simulink model "title4"  (R2024b)
settings: Solver=VariableStepAuto  StartTime=0.0  StopTime=2  RelTol=1e-3
libraries: fl_lib x10, spsSeriesRLCBranchLib x6, nesl_utility x5, spsThyristorLib x4, spsVoltageMeasurementLib x4, spsCurrentMeasurementLib x2, spsDiodeLib x2, spsMosfetLib x2, simulink x2, spsGroundLib x1, slpidlib x1, eePwmGenerator x1
settings Model: VariantFading=off  Creator=Abdal  LastModifiedBy=Abdal
settings DebuggingCC: AlgebraicLoopMsg=none

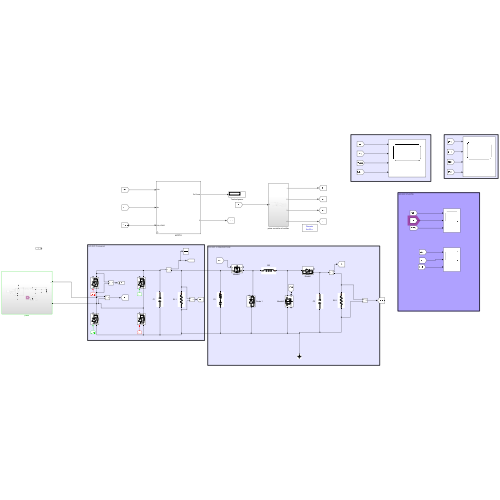
[thumbnail: Simulink's stored preview of the top-level diagram]
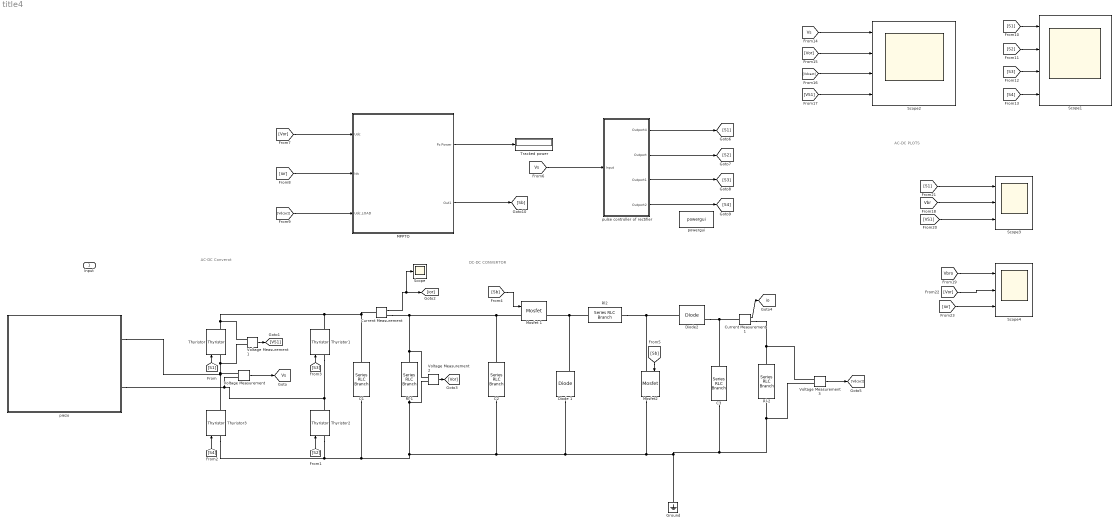
== system title4 ==
  note: AC-DC PLOTS
  note: DC-DC CONVERTOR
  note: AC-DC Converot
  Input : Inport
  C1 : spsSeriesRLCBranchLib/Series RLC Branch  LConnTagsString=__new0  RConnTagsString=__new0  BranchType=C  Resistance=1  Inductance=1e-3  SetiL0=off  InitialCurrent=0  Capacitance=4500e-6  Setx0=off  InitialVoltage=0  Measurements=None
  C2 : spsSeriesRLCBranchLib/Series RLC Branch  LConnTagsString=__new0  RConnTagsString=__new0  BranchType=RC  Resistance=1  Inductance=1e-3  SetiL0=off  InitialCurrent=0  Capacitance=1e-6  Setx0=off  InitialVoltage=0  Measurements=None
  C3 : spsSeriesRLCBranchLib/Series RLC Branch  LConnTagsString=__new0  RConnTagsString=__new0  BranchType=C  Resistance=1  Inductance=1e-3  SetiL0=off  InitialCurrent=0  Capacitance=100e-6  Setx0=off  InitialVoltage=0  Measurements=None
  Current Measurement : spsCurrentMeasurementLib/Current Measurement  PhasorSimulation=off  OutputType=Complex  PSBequivalent=0
  Current Measurement1 : spsCurrentMeasurementLib/Current Measurement  PhasorSimulation=off  OutputType=Complex  PSBequivalent=0
  "Diode 1 " : spsDiodeLib/Diode  Ron=0.001  Lon=0  Vf=0.8  IC=0  UseSnubber=0  Rs=500  Cs=250e-9  Measurements=on
  Diode2 : spsDiodeLib/Diode  Ron=0.001  Lon=0  Vf=0.8  IC=0  UseSnubber=0  Rs=500  Cs=250e-9  Measurements=on
  Ground : spsGroundLib/Ground  LConnTagsString=a
  MPPTO : Subsystem  mask{Dstep=0.01}
      mask prompts: Dstep "Perturbation step ΔD"
  "Mosfet 1 " : spsMosfetLib/Mosfet  Ron=0.1  Lon=0  Rd=0.01  Vfd=0  IC=0  Rs=1e5  Cs=inf  Measurements=on
  Mosfet2 : spsMosfetLib/Mosfet  Ron=0.1  Lon=0  Rd=0.01  Vfd=0  IC=0  Rs=1e5  Cs=inf  Measurements=on
  Rl-1 : spsSeriesRLCBranchLib/Series RLC Branch  LConnTagsString=__new0  RConnTagsString=__new0  BranchType=R  Resistance=1  Inductance=1e-3  SetiL0=off  InitialCurrent=0  Capacitance=1e-6  Setx0=off  InitialVoltage=0  Measurements=None
  Rl-2 : spsSeriesRLCBranchLib/Series RLC Branch  LConnTagsString=__new0  RConnTagsString=__new0  BranchType=R  Resistance=4000  Inductance=1e-3  SetiL0=off  InitialCurrent=0  Capacitance=1e-6  Setx0=off  InitialVoltage=0  Measurements=None
  Rl2 : spsSeriesRLCBranchLib/Series RLC Branch  LConnTagsString=__new0  RConnTagsString=__new0  BranchType=L  Resistance=1  Inductance=45e-6  SetiL0=off  InitialCurrent=0  Capacitance=1e-6  Setx0=off  InitialVoltage=0  Measurements=None
  Scope : Scope
  Scope1 : Scope  NumInputPorts=4
  Scope2 : Scope  NumInputPorts=4
  Scope3 : Scope  NumInputPorts=3
  Scope4 : Scope  NumInputPorts=3
  Thyristor : spsThyristorLib/Thyristor  Ron=100  Lon=0  Vf=0.8  IC=0  Rs=500  Cs=250e-9  Measurements=on
  Thyristor1 : spsThyristorLib/Thyristor  Ron=0.001  Lon=0  Vf=0.8  IC=0  Rs=500  Cs=250e-9  Measurements=on
  Thyristor2 : spsThyristorLib/Thyristor  Ron=0.001  Lon=0  Vf=0.8  IC=0  Rs=500  Cs=250e-9  Measurements=on
  Thyristor3 : spsThyristorLib/Thyristor  Ron=0.001  Lon=0  Vf=0.8  IC=0  Rs=500  Cs=250e-9  Measurements=on
  Tracked power : Display
  Voltage Measurement{,1..3} (4 alike) : spsVoltageMeasurementLib/Voltage Measurement  PhasorSimulation=off  OutputType=Complex  PSBequivalent=0
  piezo : Subsystem
  powergui : spspowerguiLib/powergui  Priority=1  SimulationMode=Discrete  SampleTime=50e-6  frequency=60  Iterations=50  frequencyindice=0  Pbase=100e6  ErrMax=1e-4  UnitsV=kV  UnitsW=MW  buscounter=0  FunctionMessages=off  echomessages=off  EnableUseOfTLC=off  CurrentSourceSwitches=off  DisableSnubberDevices=off  DisableRonSwitches=off  DisableVfSwitches=off  DisplayEquations=off  AutomaticDiscreteSolvers=off  SolverType=Tustin/Backward Euler (TBE)  Interpol=off  ExternalGateDelay=off  methode=off  Ts=100  x0status=blocks  SPID=on  SwTol=0  HookPort=off  NonlinearTolerance=1e-4  nMaxIteration=100  ContinueOnMaxIteration=off  RestoreLinks=warning  ResistiveCurrentMeasurement=off  Frange=[0:2:500]  Ylog=off  Xlog=on  ShowGrid=off  save=off  variable=ZData  structure=0  ZoomFFT=off  StartTime=0.0  cycles=1  DisplayStyle=1  fundamental=60  FreqAxis=off  MaxFrequency=1000  frequencyindicesteady=1  RmsSteady=1  display=off
  pulse controller of rectifier : Subsystem
  tag scope: Vs=global, io=global
  wires:
  Voltage Measurement/1 -> [Vs]
  [S1] -> Thyristor/1
  [S2] -> Thyristor2/1
  [S3] -> Thyristor1/1
  [S4] -> Thyristor3/1
  Voltage Measurement1/1 -> [VS1]
  Current Measurement/1 -> Scope/1, [ior]
  Voltage Measurement2/1 -> [Vor]
  [Sb] -> "Mosfet 1 "/1
  [Sb] -> Mosfet2/1
  Current Measurement1/1 -> [io]
  [Vs] -> pulse controller of rectifier/1(Input)
  pulse controller of rectifier/4(Outport2) -> [S4]
  MPPTO/1(Pz Power) -> Tracked power/1
  MPPTO/2(Out1) -> [Sb]
  [Vor] -> MPPTO/1(Udc)
  [ior] -> MPPTO/2(Idc)
  [Vdcact] -> MPPTO/3(Udc,LOAD)
  Voltage Measurement3/1 -> [Vdcact]
  [S1] -> Scope1/1
  [S2] -> Scope1/2
  [S3] -> Scope1/3
  [S4] -> Scope1/4
  pulse controller of rectifier/1(Outport4) -> [S1]
  pulse controller of rectifier/2(Outport) -> [S2]
  pulse controller of rectifier/3(Outport1) -> [S3]
  [Vs] -> Scope2/1
  [Vor] -> Scope2/2
  [Vdcact] -> Scope2/3
  [VS1] -> Scope2/4
  [Vbro] -> Scope4/1
  [Vor] -> Scope4/2
  [ior] -> Scope4/3
  [VS1] -> Scope3/3
  [Vbr] -> Scope3/2
  [S1] -> Scope3/1
  connections:
  Thyristor3/RConn1 -- piezo/LConn1 -- Voltage Measurement/LConn1 -- Voltage Measurement1/LConn2 -- Thyristor/LConn1
  Thyristor/RConn1 -- Voltage Measurement1/LConn1 -- Thyristor1/RConn1 -- Current Measurement/LConn1 -- C1/LConn1
  Thyristor1/LConn1 -- Voltage Measurement/LConn2 -- piezo/LConn2 -- Thyristor2/RConn1
  Thyristor3/LConn1 -- Thyristor2/LConn1 -- Voltage Measurement2/LConn2 -- Rl-1/RConn1 -- Ground/LConn1 -- C3/RConn1 -- Voltage Measurement3/LConn2 -- Rl-2/RConn1 -- Mosfet2/RConn1 -- "Diode 1 "/LConn1 -- C2/RConn1 -- C1/RConn1
  Rl2/RConn1 -- "Diode 1 "/RConn1 -- "Mosfet 1 "/RConn1
  Rl2/LConn1 -- Diode2/LConn1 -- Mosfet2/LConn1
  Diode2/RConn1 -- Current Measurement1/LConn1 -- C3/LConn1
  Current Measurement1/RConn1 -- Voltage Measurement3/LConn1 -- Rl-2/LConn1
  C2/LConn1 -- Voltage Measurement2/LConn1 -- Rl-1/LConn1 -- Current Measurement/RConn1 -- "Mosfet 1 "/LConn1

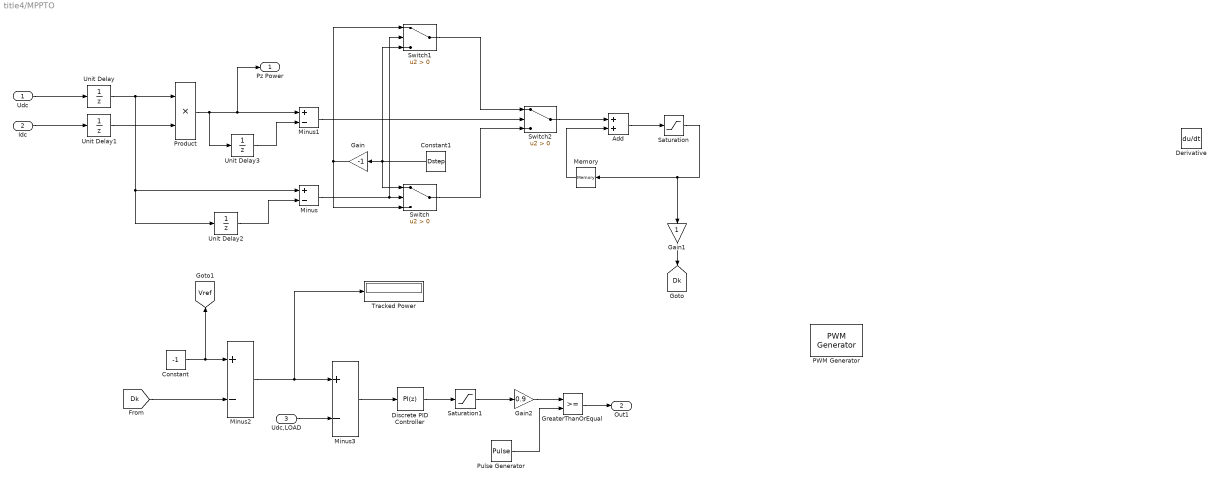
== system title4/MPPTO ==
  Udc : Inport
  Idc : Inport  Port=2
  Udc,LOAD : Inport  Port=3
  Add : Sum
  Constant : Constant  Value=-1  VectorParams1D=off
  Constant1 : Constant  Value=Dstep
  Derivative : Derivative
  Discrete PID Controller : slpidlib/PID Controller  Controller=PI  Form=Ideal  TimeDomain=Discrete-time  UseExternalTs=off  SampleTime=-1  IntegratorMethod=Forward Euler  FilterMethod=Forward Euler  ControllerParametersSource=internal  P=0.0143  I=0.0357  UseKiTs=off  D=0  UseExternalDerivativeSource=off  N=100  UseFilter=on  TunerSelectOption=Frequency Response Based  InitialConditionSource=internal  InitialConditionForIntegrator=0  InitialConditionForFilter=0  DifferentiatorICPrevScaledInput=0  ExternalReset=none  TrackingMode=off  Kt=1  LimitOutput=off  SatLimitsSource=internal  UpperSaturationLimit=inf  LowerSaturationLimit=-inf  LinearizeAsGain=off  AntiWindupMode=none  Kb=1  LimitIntegrator=off  UpperIntegratorSaturationLimit=inf  LowerIntegratorSaturationLimit=-inf  POutMin=[]  POutMax=[]  IOutMin=[]  IOutMax=[]  DOutMin=[]  DOutMax=[]  NOutMin=[]  NOutMax=[]  SumOutMin=[]  SumOutMax=[]  SaturationOutMin=[]  SaturationOutMax=[]  PParamMin=[]  PParamMax=[]  IParamMin=[]  IParamMax=[]  DParamMin=[]  DParamMax=[]  NParamMin=[]  NParamMax=[]  KbParamMin=[]  KbParamMax=[]  KtParamMin=[]  KtParamMax=[]  KbOutMin=[]  KbOutMax=[]  KtOutMin=[]  KtOutMax=[]  IntegratorOutMin=[]  IntegratorOutMax=[]  FilterOutMin=[]  FilterOutMax=[]  SumI1OutMin=[]  SumI1OutMax=[]  SumI2OutMin=[]  SumI2OutMax=[]  SumI3OutMin=[]  SumI3OutMax=[]  SumI4OutMin=[]  SumI4OutMax=[]  SumDOutMin=[]  SumDOutMax=[]  DifferentiatorOutMin=[]  DifferentiatorOutMax=[]  FilterDiffOutCoefMin=[]  FilterDiffOutCoefMax=[]  ReciprocalOutMin=[]  ReciprocalOutMax=[]  SumDenOutMin=[]  SumDenOutMax=[]  SumNumOutMin=[]  SumNumOutMax=[]  DivideOutMin=[]  DivideOutMax=[]  UdiffTsProdOutMin=[]  UdiffTsProdOutMax=[]  NTsProdOutMin=[]  NTsProdOutMax=[]  UintegralTsProdOutMin=[]  UintegralTsProdOutMax=[]  UngainTsProdOutMin=[]  UngainTsProdOutMax=[]  ClampingZeroOutDataTypeStr=Inherit: Inherit via back propagation  ClampingZeroOutMin=[]  ClampingZeroOutMax=[]  FilterDenConstantOutDataTypeStr=Inherit: Inherit via back propagation  FilterDenConstantOutMin=[]  FilterDenConstantOutMax=[]  PCopyOutDataTypeStr=Inherit: Inherit via back propagation  PCopyOutMin=[]  PCopyOutMax=[]  NCopyOutDataTypeStr=Inherit: Inherit via back propagation  NCopyOutMin=[]  NCopyOutMax=[]  IntegratorContinuousStateAttributes=''  IntegratorStateMustResolveToSignalObject=off  IntegratorRTWStateStorageClass=Auto  FilterContinuousStateAttributes=''  FilterStateMustResolveToSignalObject=off  FilterRTWStateStorageClass=Auto  ParallelPVariant=Passthrough  IdealPVariant=InternalParameters  IVariant=InternalParameters  DVariant=Disabled  IntegratorVariant=Discrete  SatVariant=Disabled  AWVariant=Passthrough  PCopyVariant=Disabled  TRVariant=Disabled  FdbkBlocksVariant=Forward  IdealPFdbkVariant=Disabled  SatFdbkVariant=Disabled  DerivativeFilterVariant=Disabled  NVariant=Disabled  NCopyVariant=Disabled_SignalSpec  FilterICVariant=Disabled  IntegratorICVariant=InternalICs  ExternalResetVariant=Disabled  TRSumVariant=Passthrough  SumFdbkVariant=Disabled  SumVariant=Sum_PI  TsampFilterVariant=InternalTs  TsampNgainVariant=Passthrough  TsampIntegralVariant=Disabled_SignalSpec  ExternalSaturationOutDataTypeStr=Inherit: Same as second input  DerivativeSourceVariant=Disabled  PreIntVariant=InternalPreInt
      settings: LibrarySourceBlock=simulink/Discrete/Discrete PID Controller
  Gain : Gain  Gain=-1
  Gain1 : Gain
  Gain2 : Gain  Gain=0.9
  GreaterThanOrEqual : RelationalOperator  OutDataTypeStr=boolean  RndMeth=Simplest  InputSameDT=off
  Memory : Memory
  Minus{,1..3} (4 alike) : Sum  Inputs=+-
  PWM Generator : eePwmGenerator/PWM Generator  CarrCount=Up  Tper=0.001  Tdelay=0  Ts=5e-5
  Product : Product
  Pulse Generator : DiscretePulseGenerator  PulseType=Time based  Period=0.00005  PulseWidth=50
  Saturation : Saturate  UpperLimit=0.6  LowerLimit=0.4
  Saturation1 : Saturate  UpperLimit=0.6  LowerLimit=0.4
  Switch : Switch  Criteria=u2 > Threshold  SaturateOnIntegerOverflow=off  InputSameDT=off
  Switch1 : Switch  Criteria=u2 > Threshold  SaturateOnIntegerOverflow=off  InputSameDT=off
  Switch2 : Switch  Criteria=u2 > Threshold  SaturateOnIntegerOverflow=off  InputSameDT=off
  Tracked Power : Display
  Unit Delay{,1..3} (4 alike) : UnitDelay  SampleTime=-1  HasFrameUpgradeWarning=on
  Pz Power : Outport
  Out1 : Outport  Port=2
  tag scope: Dk=global, Vref=global
  wires:
  Udc/1 -> Unit Delay/1
  Idc/1 -> Unit Delay1/1
  Unit Delay/1 -> Product/1, Minus/1, Unit Delay2/1
  Unit Delay1/1 -> Product/2
  Unit Delay2/1 -> Minus/2
  Minus/1 -> Switch1/2, Switch/2
  Unit Delay3/1 -> Minus1/2
  Minus1/1 -> Switch2/2
  Switch1/1 -> Switch2/1
  Switch/1 -> Switch2/3
  Switch2/1 -> Add/1
  Add/1 -> Saturation/1
  Gain/1 -> Switch/3, Switch1/1
  Saturation/1 -> Gain1/1, Memory/1
  Memory/1 -> Add/2
  Constant1/1 -> Switch/1, Switch1/3, Gain/1
  Gain1/1 -> [Dk]
  Product/1 -> Unit Delay3/1, Pz Power/1, Minus1/1
  [Dk] -> Minus2/2
  Constant/1 -> Minus2/1, [Vref]
  Minus2/1 -> Tracked Power/1, Minus3/1
  Udc,LOAD/1 -> Minus3/2
  Minus3/1 -> Discrete PID Controller/1
  Discrete PID Controller/1 -> Saturation1/1
  Saturation1/1 -> Gain2/1
  Gain2/1 -> GreaterThanOrEqual/1
  Pulse Generator/1 -> GreaterThanOrEqual/2
  GreaterThanOrEqual/1 -> Out1/1

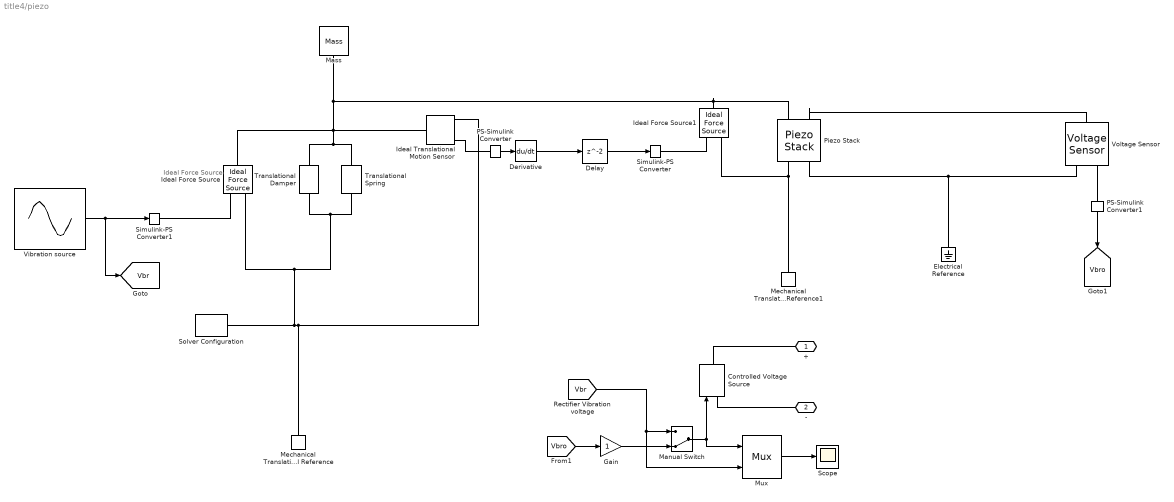
== system title4/piezo ==
  note: Ideal Force Source
  Controlled Voltage Source : spsControlledVoltageSourceLib/Controlled Voltage Source  Initialize=on  Source_Type=AC  Amplitude=0  Phase=0  Frequency=5000  Measurements=None
  Delay : Delay
  Derivative : Derivative
  Electrical Reference : fl_lib/Electrical/Electrical Elements/Electrical Reference
  Gain : Gain
  Ideal Force Source : fl_lib/Mechanical/Mechanical Sources/Ideal Force Source
  Ideal Force Source1 : fl_lib/Mechanical/Mechanical Sources/Ideal Force Source
  Ideal Translational Motion Sensor : fl_lib/Mechanical/Mechanical Sensors/Ideal Translational Motion Sensor  reference=foundation.enum.MeasurementReference.difference  acceleration_port=false  velocity_port=true  position_port=true  offset=0 m
  Manual Switch : ManualSwitch  CurrentSetting=0
  Mass : fl_lib/Mechanical/Translational Elements/Mass  mass=3.6 kg  num_ports=foundation.enum.numPorts2.one  v_specify=off  v_priority=High  v=0 m/s  v_nominal_specify=off  v_nominal_value=1  v_nominal_unit=m/s  f_specify=off  f_priority=None  f=0 N  f_nominal_specify=off  f_nominal_value=1  f_nominal_unit=N
  Mechanical Translational Reference : fl_lib/Mechanical/Translational Elements/Mechanical Translational Reference
  Mechanical Translational Reference1 : fl_lib/Mechanical/Translational Elements/Mechanical Translational Reference
  Mux : Mux  Inputs=2
      settings: DisplayOption=signals
  PS-Simulink Converter : nesl_utility/PS-Simulink Converter  PhysicalDomain=network_engine_domain  SubClassName=ps_output  LeftPortType=input  RightPortType=output  PseudoPeriodic=off  Frequencies=[]  VectorFormat=inherit  Unit=inherit  AffineConversion=off
  PS-Simulink Converter1 : nesl_utility/PS-Simulink Converter  PhysicalDomain=network_engine_domain  SubClassName=ps_output  LeftPortType=input  RightPortType=output  PseudoPeriodic=off  Frequencies=[]  VectorFormat=inherit  Unit=inherit  AffineConversion=off
  Piezo Stack : ee_lib/Electromechanical/Mechatronic Actuators/Piezo Stack  param=ee.enum.actuators.datasheetOrMaterialProps.datasheet  A=100 mm^2  L0=36 mm  dt=0.3 mm  NL=50  dL0=0.038 mm  F0=3800 N  V0=120 V  C0=13 uF  d=500e-12 m/V  epsilon=2.1240e-08 F/m  s=19e-12 m^2/N  paramDyn=ee.enum.actuators.datasheetOrMaterialProps.datasheet  f=inf kHz  Qm=inf  Mass=0 g  lam=0 N*s/m  force_specify=off  force_priority=None  force=0 N  force_nominal_specify=off  force_nominal_value=1  force_nominal_unit=N  vel_specify=off  vel_priority=None  vel=0 mm/s  vel_nominal_specify=off  vel_nominal_value=1  vel_nominal_unit=mm/s  x_specify=off  x_priority=None  x=0 mm  x_nominal_specify=off  x_nominal_value=1  x_nominal_unit=mm  v_specify=off  v_priority=None  v=0 V  v_nominal_specify=off  v_nominal_value=1  v_nominal_unit=V
      settings: InternalSimscapePortConfiguration="{\"Bottom\":[],\"Left\":[{\"id\":\"p\",\"label\":\"+\",\"type\":\"foundation.electrical.electrical\"},{\"id\":\"R\",\"label\":\"R\",\"type\":\"foundation.mechanical.translational.translational\"}],\"Right\":[{\"id\":\"n\",\"label\":\"-\",\"type\":\"foundation.electrical.electrical\"},{\"id\":\"C\",\"label\":\"C\",\"type\":\"foundation.mechanical.translational.translational\"}],\"Top\":[]}"
  Scope : Scope
  Simulink-PS Converter : nesl_utility/Simulink-PS Converter  PhysicalDomain=network_engine_domain  SubClassName=ps_input  LeftPortType=input  RightPortType=output  PseudoPeriodic=off  Frequencies=[]  NoiseDistribution=none  NoiseParameters=[]  Unit=1  AffineConversion=off  FilteringAndDerivatives=provide  SimscapeFilterOrder=1  InputFilterTimeConstant=0.001  UdotUserProvided=0
  Simulink-PS Converter1 : nesl_utility/Simulink-PS Converter  PhysicalDomain=network_engine_domain  SubClassName=ps_input  LeftPortType=input  RightPortType=output  PseudoPeriodic=off  Frequencies=[]  NoiseDistribution=none  NoiseParameters=[]  Unit=1  AffineConversion=off  FilteringAndDerivatives=provide  SimscapeFilterOrder=1  InputFilterTimeConstant=0.001  UdotUserProvided=0
  Solver Configuration : nesl_utility/Solver Configuration  PhysicalDomain=network_engine_domain  SubClassName=solver  LeftPortType=input  RightPortType=generic  Tones=[]  Harmonics=[]  SimulateNoise=off  Profile=off  UseLocalSampling=off  EnableSwitchedLinearOptims=on  FrequencyDomain=off  UseCCode=off  RelTol=0.001  AbsTol=0.001  MinStep=1e-09  ToWorkspace=off  RevertToSquareIcSolve=off  NumHomotopyIterations=100  PhasorMode=off  PhasorModeNumHarmonics=1  ConsistencySolver=NEWTON_XTOL_AFTER_FTOL  IndexReductionMethod=DerivativeReplacement  DoDC=off  ResidualTolerance=1e-09  ConsistencyTolSource=GLOBAL  ConsistencyAbsTol=0.001  ConsistencyRelTol=0.001  ConsistencyTolFactor=0.001  UseLocalSolver=off  LocalSolverChoice=NE_BACKWARD_EULER_ADVANCER  ResolveIndetEquations=on  FunctionEvalNumThread=1  LocalSolverSampleTime=0.001  DoFixedCost=off  MaxNonlinIter=3  MaxModeIter=2  ComputeImpulses=off  ImpulseIterations=2  LinearAlgebra=auto  LinearAlgebraNumThread=0  EquationFormulation=NE_TIME_EF  DelaysMemoryBudget=1024  AutomaticFiltering=on  FilteringTimeConstant=0.001  PartitionStorageMethod=AS_NEEDED  PartitionMemoryBudget=1024  PartitionMethod=ROBUST  MultibodyUseLocalSolver=off  MultibodyLocalSolverChoice=ODE1  MultibodyLocalSolverSampleTime=0.001
  Translational Damper : fl_lib/Mechanical/Translational Elements/Translational Damper  D=100 N*s/m  v_specify=off  v_priority=None  v=0 m/s  v_nominal_specify=off  v_nominal_value=1  v_nominal_unit=m/s  f_specify=off  f_priority=None  f=0 N  f_nominal_specify=off  f_nominal_value=1  f_nominal_unit=N
  Translational Spring : fl_lib/Mechanical/Translational Elements/Translational Spring  spr_rate=400 N/m  v_specify=off  v_priority=None  v=0 m/s  v_nominal_specify=off  v_nominal_value=1  v_nominal_unit=m/s  f_specify=off  f_priority=None  f=0 N  f_nominal_specify=off  f_nominal_value=1  f_nominal_unit=N  x_specify=off  x_priority=High  x=0 m  x_nominal_specify=off  x_nominal_value=1  x_nominal_unit=m
  Vibration source : Sin  Amplitude=150  Frequency=50  SampleTime=0
  Voltage Sensor : fl_lib/Electrical/Electrical Sensors/Voltage Sensor
  + : PMIOPort  Side=Left
  - : PMIOPort  Port=2  Side=Left
  tag scope: Vbr=global, Vbro=global
  wires:
  PS-Simulink Converter/1 -> Derivative/1
  Derivative/1 -> Delay/1
  Vibration source/1 -> [Vbr], Simulink-PS Converter1/1
  PS-Simulink Converter1/1 -> [Vbro]
  [Vbro] -> Gain/1
  Manual Switch/1 -> Mux/1, Controlled Voltage Source/1
  [Vbr] -> Mux/2, Manual Switch/1
  Gain/1 -> Manual Switch/2
  Mux/1 -> Scope/1
  Delay/1 -> Simulink-PS Converter/1
  connections:
  Translational Damper/LConn1 -- Piezo Stack/LConn2 -- Ideal Force Source1/LConn1 -- Mass/LConn1 -- Ideal Force Source/LConn1 -- Ideal Translational Motion Sensor/LConn1 -- Translational Spring/LConn1
  Translational Damper/RConn1 -- Ideal Translational Motion Sensor/RConn1 -- Mechanical Translational Reference/LConn1 -- Solver Configuration/RConn1 -- Ideal Force Source/RConn2 -- Translational Spring/RConn1
  Mechanical Translational Reference1/LConn1 -- Ideal Force Source1/RConn2 -- Piezo Stack/RConn2
  Piezo Stack/LConn1 -- Voltage Sensor/LConn1
  Piezo Stack/RConn1 -- Electrical Reference/LConn1 -- Voltage Sensor/RConn2
  PS-Simulink Converter/LConn1 -- Ideal Translational Motion Sensor/RConn3
  Simulink-PS Converter/RConn1 -- Ideal Force Source1/RConn1
  Simulink-PS Converter1/RConn1 -- Ideal Force Source/RConn1
  PS-Simulink Converter1/LConn1 -- Voltage Sensor/RConn1
  Controlled Voltage Source/RConn1 -- +/RConn1
  Controlled Voltage Source/LConn1 -- -/RConn1

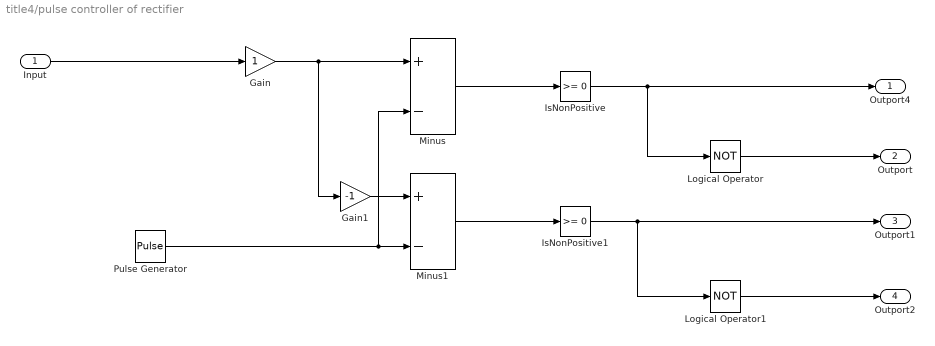
== system title4/pulse controller of rectifier ==
  Input : Inport
  Gain : Gain
  Gain1 : Gain  Gain=-1
  IsNonPositive : simulink/Logic and Bit Operations/Compare To Zero  relop=>=  OutDataTypeStr=boolean
      settings: LibrarySourceBlock=|
      | simulink/Quick Insert/Logic and Bit
      | Operations/IsNonPositive
  IsNonPositive1 : simulink/Logic and Bit Operations/Compare To Zero  relop=>=  OutDataTypeStr=boolean
      settings: LibrarySourceBlock=|
      | simulink/Quick Insert/Logic and Bit
      | Operations/IsNonPositive
  Logical Operator : Logic  Operator=NOT  AllPortsSameDT=off  OutDataTypeStr=boolean
  Logical Operator1 : Logic  Operator=NOT  AllPortsSameDT=off  OutDataTypeStr=boolean
  Minus : Sum  Inputs=+-
  Minus1 : Sum  Inputs=+-
  Pulse Generator : DiscretePulseGenerator  PulseType=Time based  Period=0.0002  PulseWidth=50
  Outport4 : Outport
  Outport : Outport  Port=2
  Outport1 : Outport  Port=3
  Outport2 : Outport  Port=4
  wires:
  Gain/1 -> Gain1/1, Minus/1
  Gain1/1 -> Minus1/1
  Pulse Generator/1 -> Minus/2, Minus1/2
  Minus/1 -> IsNonPositive/1
  Minus1/1 -> IsNonPositive1/1
  IsNonPositive/1 -> Outport4/1, Logical Operator/1
  IsNonPositive1/1 -> Outport1/1, Logical Operator1/1
  Logical Operator/1 -> Outport/1
  Logical Operator1/1 -> Outport2/1
  Input/1 -> Gain/1
